simulink library "sm_car_scene_double_lane_change"  (R2024b)
settings: Solver=VariableStepAuto  StartTime=0.0  StopTime=10.0  RelTol=1e-3
undefined symbols (not defined in the file or in its folder): Scene, X, Y, Z
libraries: Scene_Utilities x3, sm_lib x2
Description:
  | Scene of Simscape Vehicle Templates Library
  | 
  | Copyright 2018-2024 The MathWorks, Inc.
settings Model: Creator=smiller  LastModifiedBy=smiller
settings SolverCC: AlgebraicLoopSolver=TrustRegion
settings DataIOCC: ReturnWorkspaceOutputs=off
settings OptimizationCC: ReuseModelBlockBuffer=off
settings DebuggingCC: UnconnectedInputMsg=warning  UnconnectedOutputMsg=warning  UnconnectedLineMsg=warning  ArithmeticOperatorsInVariantConditions=warning
settings ModelReferenceCC: EnableRefExpFcnMdlSchedulingChecks=on
settings SFSimCC: CustomCodeUndefinedFunction=UseInterfaceOnly
settings RTWCC: GPUComputeCapability=3.5  DLArmComputeVersion=19.05

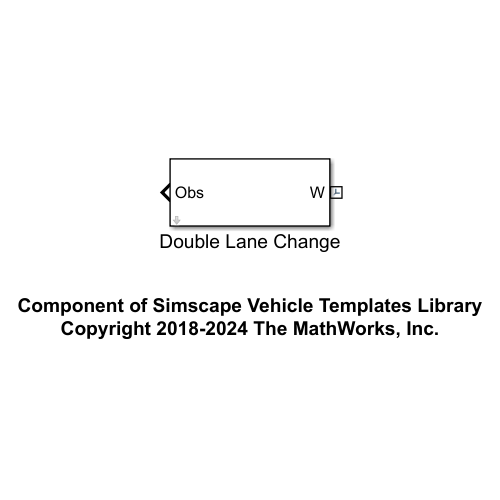
[thumbnail: Simulink's stored preview of the top-level diagram]
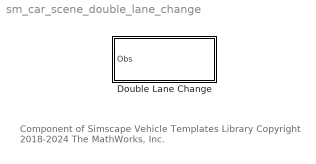
== system sm_car_scene_double_lane_change ==
  note: Component of Simscape Vehicle Templates Library
      | Copyright 2018-2024 The MathWorks, Inc.
  Double Lane Change : Subsystem  mask{road=Scene.Double_Lane_Change.Road, dashes=Scene.Double_Lane_Change.Dashes, cones=Scene.Double_Lane_Change.Cones}
      mask prompts: road "Road (structure)"; dashes "Dashes (structure)"; cones "Cones (structure)"

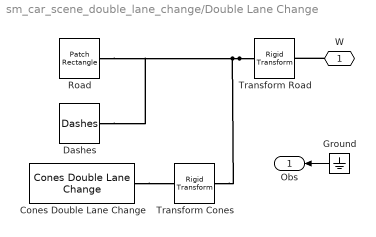
== system sm_car_scene_double_lane_change/Double Lane Change ==
  Cones Double Lane Change : Scene_Utilities/Cones Double Lane Change  lane_width=cones.lane_width  lane_separation=cones.lane_lateral_offset  start_lane_a=cones.lane_a_offset  A1_to_A5=cones.lane_a_length  A_to_B_x=cones.gap_a_to_b  B1_to_B5=cones.lane_b_length  B_to_C_x=cones.gap_b_to_c  C1_to_C5=cones.lane_c_length  height=cones.height  baseThickness=cones.base_thickness  baseWidth=cones.base_width  coneBaseDiameter=cones.bottom_diameter  coneTopDiameter=cones.top_diameter  reflectiveStripHeight=cones.strip_height  coneColor=cones.clr  reflectiveStripColor=cones.strip_clr
  Dashes : Scene_Utilities/Dashes  dash_pitch=dashes.pitch  num_dashes=dashes.num  dash_l=dashes.l  dash_h=dashes.h  dash_w=dashes.w  thickness_base=dashes.base_h  dash_clr=dashes.clr  dash_opc=dashes.opc
  Ground : Ground
  Road : Scene_Utilities/Patch Rectangle  gp_l=road.l  gp_w=road.w  gp_h=road.h  gp_clr=road.clr  gp_opc=road.opc
  Transform Cones : sm_lib/Frames and Transforms/Rigid Transform  RotationMethod=None  FollAlignAxisA=+X  BaseAlignAxisA=+Y  FollAlignAxisB=+Y  BaseAlignAxisB=+Z  RotationStandardAxis=+Z  RotationAngle=0.0  RotationAngleUnits=deg  RotationArbitraryAxis=[0 0 1]  RotationSequenceAxes=FollowerAxes  RotationSequence=XYX  RotationSequenceAngles=[0 0 0]  RotationSequenceAnglesUnits=deg  RotationMatrix=[1 0 0; 0 1 0; 0 0 1]  Quaternion=[1 0 0 0]  TranslationMethod=StandardAxis  TranslationCartesianOffset=[0 0 0]  TranslationCartesianOffsetUnits=m  TranslationStandardAxis=-X  TranslationStandardOffset=road.l/2  TranslationStandardOffsetUnits=m  TranslationROffset=0  TranslationROffsetUnits=m  TranslationThetaOffset=0  TranslationThetaOffsetUnits=deg  TranslationZOffset=0  TranslationZOffsetUnits=m
  Transform Road : sm_lib/Frames and Transforms/Rigid Transform  RotationMethod=RotationSequence  FollAlignAxisA=+X  BaseAlignAxisA=+Y  FollAlignAxisB=+Y  BaseAlignAxisB=+Z  RotationStandardAxis=+Z  RotationAngle=0.0  RotationAngleUnits=deg  RotationArbitraryAxis=[0 0 1]  RotationSequenceAxes=BaseAxes  RotationSequence=ZYX  RotationSequenceAngles=[road.yaw road.pitch road.roll]  RotationSequenceAnglesUnits=rad  RotationMatrix=[1 0 0; 0 1 0; 0 0 1]  Quaternion=[1 0 0 0]  TranslationMethod=Cartesian  TranslationCartesianOffset=[road.x road.y road.z]  TranslationCartesianOffsetUnits=m  TranslationStandardAxis=+Z  TranslationStandardOffset=0  TranslationStandardOffsetUnits=m  TranslationROffset=0  TranslationROffsetUnits=m  TranslationThetaOffset=0  TranslationThetaOffsetUnits=deg  TranslationZOffset=0  TranslationZOffsetUnits=m
  W : PMIOPort  Side=Left
  Obs : Outport  VectorParamsAs1DForOutWhenUnconnected=off
  wires:
  Ground/1 -> Obs/1
  connections:
  Cones Double Lane Change/LConn1 -- Transform Cones/RConn1
  Transform Road/RConn1 -- Transform Cones/LConn1 -- Road/RConn1 -- Dashes/LConn1
  W/RConn1 -- Transform Road/LConn1
